simulink model "PV_BESS_EMS"  (R2025b)
settings: Solver=VariableStepAuto  StartTime=0.0  StopTime=168  RelTol=1e-3
model workspace (MAT data in the model file):
  SOC_initial = 0.25
settings Model: Creator=raysu  LastModifiedBy=raysu

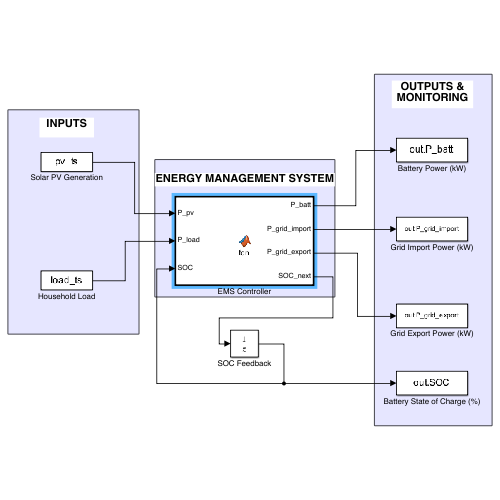
[thumbnail: Simulink's stored preview of the top-level diagram]
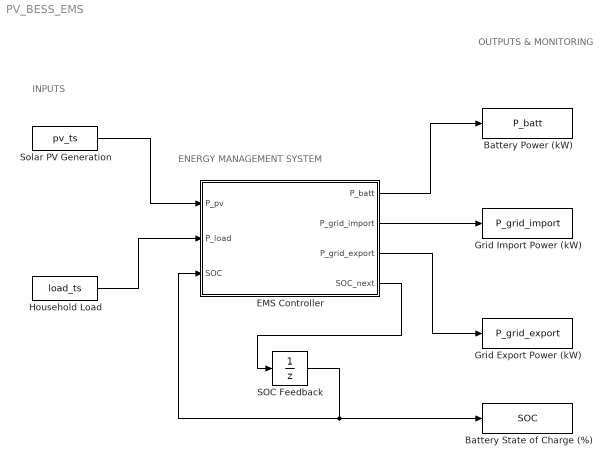
== system PV_BESS_EMS ==
  note: ENERGY MANAGEMENT SYSTEM
  note: INPUTS
  note: OUTPUTS & MONITORING
  Battery Power (kW) : ToWorkspace  VariableName=P_batt  SaveFormat=Timeseries  SampleTime=-1
  Battery State of Charge (%) : ToWorkspace  VariableName=SOC  SaveFormat=Timeseries  SampleTime=-1
  EMS Controller : MATLAB Function  TreatAsAtomicUnit=on
  Grid Export Power (kW) : ToWorkspace  VariableName=P_grid_export  SaveFormat=Timeseries  SampleTime=-1
  Grid Import Power (kW) : ToWorkspace  VariableName=P_grid_import  SaveFormat=Timeseries  SampleTime=-1
  Household Load : FromWorkspace  VariableName=load_ts
  SOC Feedback : UnitDelay  InitialCondition=SOC_initial  SampleTime=0.25  HasFrameUpgradeWarning=on
  Solar PV Generation : FromWorkspace  VariableName=pv_ts
  wires:
  Solar PV Generation/1 -> EMS Controller/1(P_pv)
  Household Load/1 -> EMS Controller/2(P_load)
  EMS Controller/4(SOC_next) -> SOC Feedback/1
  EMS Controller/1(P_batt) -> Battery Power (kW)/1
  SOC Feedback/1 -> EMS Controller/3(SOC), Battery State of Charge (%)/1
  EMS Controller/3(P_grid_export) -> Grid Export Power (kW)/1
  EMS Controller/2(P_grid_import) -> Grid Import Power (kW)/1

== matlab function PV_BESS_EMS/EMS Controller ==
  data: P_pv input; P_batt output; P_load input; SOC input; P_grid_import output; P_grid_export output; SOC_next output
function [P_batt, P_grid_import, P_grid_export, SOC_next] = ...
    fcn(P_pv, P_load, SOC)
%#codegen

% Battery parameters
E_batt = 10;             % Battery capacity (kWh)
P_charge_max = 3;        % Maximum charging power (kW)
P_discharge_max = 3;     % Maximum discharging power (kW)
SOC_min = 0.20;          % Minimum state of charge
SOC_max = 0.95;          % Maximum state of charge
eta = 0.95;              % Battery efficiency
dt = 0.25;               % Simulation time step (hour)

% Calculate net PV power
P_net = P_pv - P_load;

% Initialize outputs
P_batt = 0;
P_grid_import = 0;
P_grid_export = 0;
SOC_next = SOC;

if P_net >= 0

    % PV generation exceeds demand
    surplus = P_net;

    % Maximum power the battery can accept
    available_capacity_power = ...
        max(0, (SOC_max - SOC) * E_batt / (eta * dt));

    % Charge battery using available PV surplus
    P_charge = min(surplus, P_charge_max);
    P_charge = min(P_charge, available_capacity_power);

    % Positive battery power means charging
    P_batt = P_charge;

    % Export any remaining surplus
    P_grid_export = max(0, surplus - P_charge);

    % Update battery SOC
    SOC_next = SOC + eta * P_charge * dt / E_batt;

else

    % Demand exceeds PV generation
    deficit = -P_net;

    % Maximum power available from the battery
    available_discharge_power = ...
        max(0, (SOC - SOC_min) * E_batt * eta / dt);

    % Discharge battery to cover the deficit
    P_discharge = min(deficit, P_discharge_max);
    P_discharge = min(P_discharge, available_discharge_power);

    % Negative battery power means discharging
    P_batt = -P_discharge;

    % Import any remaining deficit from the grid
    P_grid_import = max(0, deficit - P_discharge);

    % Update battery SOC
    SOC_next = SOC - P_discharge * dt / (eta * E_batt);

end

% Enforce SOC limits
SOC_next = min(max(SOC_next, SOC_min), SOC_max);

end
